simulink model "XY_2_pen_ros2"  (R2024b)
settings: Solver=ode4  StartTime=0.0  StopTime=T_run_ros  FixedStep=Ts_ctrl  RelTol=1e-3
StopFcn:
  | XY_stop
values from neighbouring files (symbols this model uses):
  d_reach = 0.03    [XY_setup.m]
  db_v = 47    [XY_setup.m]
  db_w = 20    [XY_setup.m]
  K_c = 0    [XY_setup.m]
  K_ci = 0    [XY_setup.m]
  K_dist = 1.0    (= 1)    [XY_setup.m]
  K_ptheta = 1.4    [XY_setup.m]
  K_px = 0.3    [XY_setup.m]
  K_py = 5.0    (= 5)    [XY_setup.m]
  K_yaw = 2.0    (= 2)    [XY_setup.m]
  line_post = 0.04    [XY_setup.m]
  line_pre = 0.06    [XY_setup.m]
  pen_A = [-0.70; 0.30]    [XY_setup.m]
  pen_B = [ 0.50; 0.30]    [XY_setup.m]
  pen_d = r_pen0 - r_tag    [XY_setup.m]
  psi0 = pi/2    (= 1.57079632679)    [XY_setup.m]
  r_tag = [-0.080;  0.060]    [XY_setup.m]
  stage_c = stage_travel/2    (= 50.8)    [XY_setup.m]
  stage_travel = 101.6    [XY_setup.m]
  stage_vcmd = 0.8*stage_vmax    (= 83.2)    [XY_setup.m]
  tau_pred = 0    [XY_setup.m]
  th_tol = deg2rad(1)    [XY_setup.m]
  Ts_ctrl = 0.01    [XY_setup.m]
  v_full = 0.20    (= 0.2)    [XY_setup.m]
  v_max = 0.20    (= 0.2)    [XY_setup.m]
  v_ref = 0.03    [XY_setup.m]
  w_full = 2*k_pwm*(400 - db_w)/B_eff    (= 1.36936936937)    [XY_setup.m]
  w_max = deg2rad(45)    [XY_setup.m]
  x = c(1) + s(1)/2*[-1 1 1 -1 -1 1 1 -1]    [XY_animate.m]
  y = c(2) + s(2)/2*[-1 -1 1 1 -1 -1 1 1]    [XY_animate.m]    (also in build_xy_models.m = q(2))
  zk_xsign = -1    [XY_setup.m]
libraries: ros2lib x8, simulink x4
settings Model: Creator=admin  LastModifiedBy=admin
settings DataIOCC: ReturnWorkspaceOutputs=off

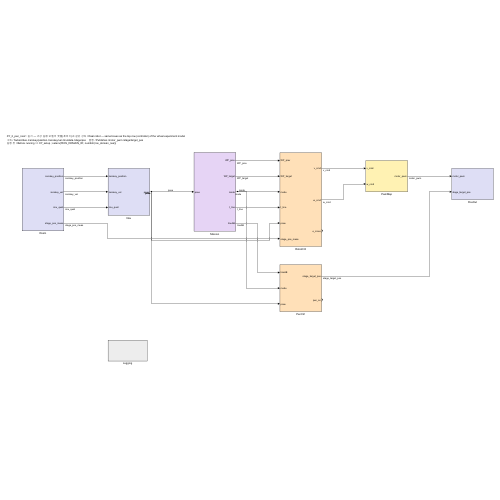
[thumbnail: Simulink's stored preview of the top-level diagram]
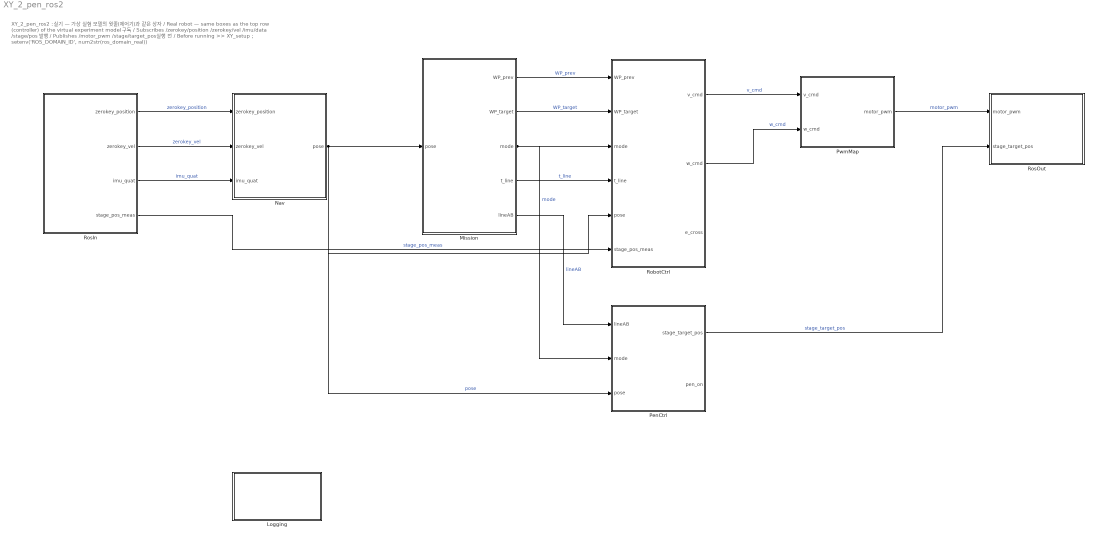
== system XY_2_pen_ros2 ==
  note: XY_2_pen_ros2 : 실기 — 가상 실험 모델의 윗줄(제어기)과 같은 상자 / Real robot — same boxes as the top row (controller) of the virtual experiment model
      | 구독 / Subscribes /zerokey/position /zerokey/vel /imu/data /stage/pos    발행 / Publishes /motor_pwm /stage/target_pos
      | 실행 전 / Before running >> XY_setup ; setenv('ROS_DOMAIN_ID', num2str(ros_domain_real))
  Logging : Subsystem
  Mission : Subsystem
  Nav : Subsystem
  PenCtrl : Subsystem
  PwmMap : Subsystem
  RobotCtrl : Subsystem
  RosIn : Subsystem
  RosOut : Subsystem
  wires:
  Nav/1(pose) -> Mission/1(pose), PenCtrl/3(pose), RobotCtrl/5(pose)  "pose"
  RosIn/1(zerokey_position) -> Nav/1(zerokey_position)  "zerokey_position"
  RosIn/2(zerokey_vel) -> Nav/2(zerokey_vel)  "zerokey_vel"
  RosIn/3(imu_quat) -> Nav/3(imu_quat)  "imu_quat"
  Mission/5(lineAB) -> PenCtrl/1(lineAB)  "lineAB"
  Mission/3(mode) -> PenCtrl/2(mode), RobotCtrl/3(mode)  "mode"
  RobotCtrl/1(v_cmd) -> PwmMap/1(v_cmd)  "v_cmd"
  RobotCtrl/2(w_cmd) -> PwmMap/2(w_cmd)  "w_cmd"
  Mission/1(WP_prev) -> RobotCtrl/1(WP_prev)  "WP_prev"
  Mission/2(WP_target) -> RobotCtrl/2(WP_target)  "WP_target"
  Mission/4(t_line) -> RobotCtrl/4(t_line)  "t_line"
  RosIn/4(stage_pos_meas) -> RobotCtrl/6(stage_pos_meas)  "stage_pos_meas"
  PwmMap/1(motor_pwm) -> RosOut/1(motor_pwm)  "motor_pwm"
  PenCtrl/1(stage_target_pos) -> RosOut/2(stage_target_pos)  "stage_target_pos"

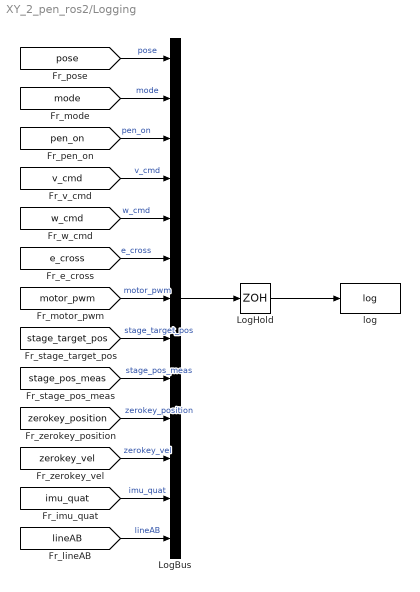
== system XY_2_pen_ros2/Logging ==
  LogBus : BusCreator  Inputs=13
  LogHold : ZeroOrderHold  Description=이산: 기록 주기 (제어기 주기와 같다) / Discrete: logging period (same as the controller period)  SampleTime=Ts_ctrl
  log : ToWorkspace  VariableName=log  SaveFormat=Timeseries  SampleTime=Ts_ctrl
  wires:
  [pose] -> LogBus/1  "pose"
  [mode] -> LogBus/2  "mode"
  [pen_on] -> LogBus/3  "pen_on"
  [v_cmd] -> LogBus/4  "v_cmd"
  [w_cmd] -> LogBus/5  "w_cmd"
  [e_cross] -> LogBus/6  "e_cross"
  [motor_pwm] -> LogBus/7  "motor_pwm"
  [stage_target_pos] -> LogBus/8  "stage_target_pos"
  [stage_pos_meas] -> LogBus/9  "stage_pos_meas"
  [zerokey_position] -> LogBus/10  "zerokey_position"
  [zerokey_vel] -> LogBus/11  "zerokey_vel"
  [imu_quat] -> LogBus/12  "imu_quat"
  [lineAB] -> LogBus/13  "lineAB"
  LogBus/1 -> LogHold/1
  LogHold/1 -> log/1

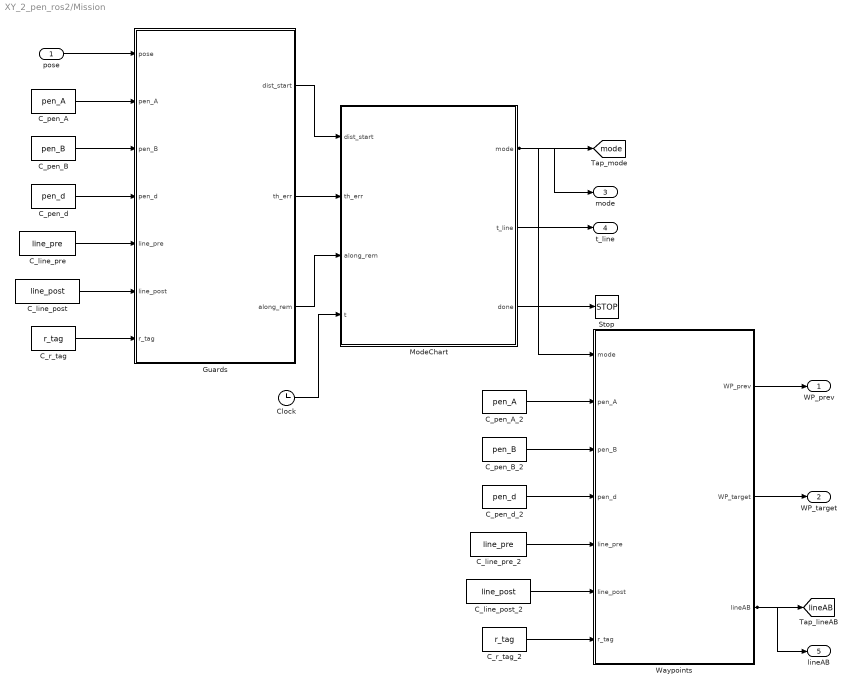
== system XY_2_pen_ros2/Mission ==
  pose : Inport
  C_line_post : Constant  Value=line_post
  C_line_post_2 : Constant  Value=line_post
  C_line_pre : Constant  Value=line_pre
  C_line_pre_2 : Constant  Value=line_pre
  C_pen_A : Constant  Value=pen_A
  C_pen_A_2 : Constant  Value=pen_A
  C_pen_B : Constant  Value=pen_B
  C_pen_B_2 : Constant  Value=pen_B
  C_pen_d : Constant  Value=pen_d
  C_pen_d_2 : Constant  Value=pen_d
  C_r_tag : Constant  Value=r_tag
  C_r_tag_2 : Constant  Value=r_tag
  Clock : Clock
  Guards : MATLAB Function  TreatAsAtomicUnit=on
  ModeChart : Stateflow chart  Description=이산: 모드는 사건 상태 (6WP_sim Chart 와 같은 역할). 전이: 거리 < d_reach, 1 s 뒤 각 오차 < th_tol, 남은 거리 < d_reach, 정지 2 s / Discrete: the mode is an event state (same role as the 6WP_sim Chart). Transitions: distance < d_reach, angle error < th_tol after 1 s, remaining distance < d_reach, stop 2 s  TreatAsAtomicUnit=on
  Stop : Stop
  Waypoints : MATLAB Function  TreatAsAtomicUnit=on
  WP_prev : Outport
  WP_target : Outport  Port=2
  mode : Outport  Port=3
  t_line : Outport  Port=4
  lineAB : Outport  Port=5
  tag scope: lineAB=global, mode=global
  wires:
  pose/1 -> Guards/1(pose)
  Clock/1 -> ModeChart/4(t)
  C_pen_A/1 -> Guards/2(pen_A)
  C_pen_d/1 -> Guards/4(pen_d)
  C_pen_B/1 -> Guards/3(pen_B)
  C_line_pre/1 -> Guards/5(line_pre)
  C_line_post/1 -> Guards/6(line_post)
  C_r_tag/1 -> Guards/7(r_tag)
  Guards/1(dist_start) -> ModeChart/1(dist_start)
  Guards/2(th_err) -> ModeChart/2(th_err)
  Guards/3(along_rem) -> ModeChart/3(along_rem)
  ModeChart/1(mode) -> Waypoints/1(mode), mode/1, [mode]
  ModeChart/2(t_line) -> t_line/1
  ModeChart/3(done) -> Stop/1
  C_pen_A_2/1 -> Waypoints/2(pen_A)
  C_pen_B_2/1 -> Waypoints/3(pen_B)
  C_pen_d_2/1 -> Waypoints/4(pen_d)
  C_line_pre_2/1 -> Waypoints/5(line_pre)
  C_line_post_2/1 -> Waypoints/6(line_post)
  C_r_tag_2/1 -> Waypoints/7(r_tag)
  Waypoints/1(WP_prev) -> WP_prev/1
  Waypoints/2(WP_target) -> WP_target/1
  Waypoints/3(lineAB) -> lineAB/1, [lineAB]

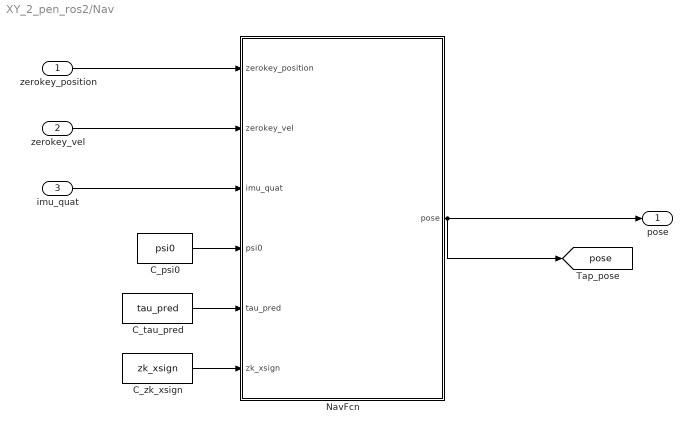
== system XY_2_pen_ros2/Nav ==
  zerokey_position : Inport
  zerokey_vel : Inport  Port=2
  imu_quat : Inport  Port=3
  C_psi0 : Constant  Value=psi0
  C_tau_pred : Constant  Value=tau_pred
  C_zk_xsign : Constant  Value=zk_xsign
  NavFcn : MATLAB Function  Description=이산: persistent (첫 요각 기억) — 구독 주기와 같다 / Discrete: persistent (stores the first yaw) — same as the subscription period  TreatAsAtomicUnit=on
  pose : Outport
  tag scope: pose=global
  wires:
  zerokey_position/1 -> NavFcn/1(zerokey_position)
  zerokey_vel/1 -> NavFcn/2(zerokey_vel)
  imu_quat/1 -> NavFcn/3(imu_quat)
  C_psi0/1 -> NavFcn/4(psi0)
  C_tau_pred/1 -> NavFcn/5(tau_pred)
  C_zk_xsign/1 -> NavFcn/6(zk_xsign)
  NavFcn/1(pose) -> pose/1, [pose]

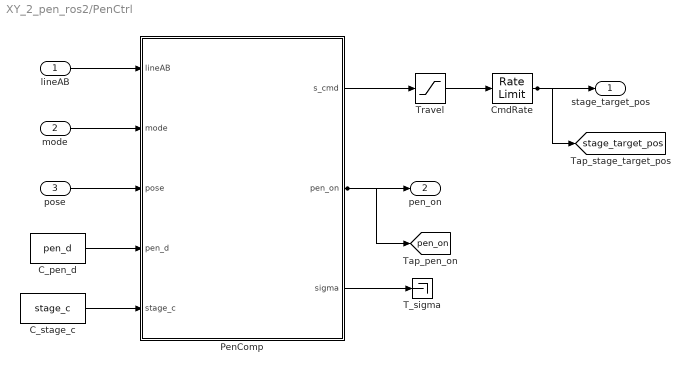
== system XY_2_pen_ros2/PenCtrl ==
  lineAB : Inport
  mode : Inport  Port=2
  pose : Inport  Port=3
  C_pen_d : Constant  Value=pen_d
  C_stage_c : Constant  Value=stage_c
  CmdRate : RateLimiter  RisingSlewLimit=stage_vcmd  FallingSlewLimit=-stage_vcmd  SampleTimeMode=inherited  InitialCondition=stage_c
  PenComp : MATLAB Function  TreatAsAtomicUnit=on
  T_sigma : Terminator
  Travel : Saturate  UpperLimit=stage_travel  LowerLimit=0
  stage_target_pos : Outport
  pen_on : Outport  Port=2
  tag scope: pen_on=global, stage_target_pos=global
  wires:
  PenComp/3(sigma) -> T_sigma/1
  lineAB/1 -> PenComp/1(lineAB)
  C_stage_c/1 -> PenComp/5(stage_c)
  C_pen_d/1 -> PenComp/4(pen_d)
  mode/1 -> PenComp/2(mode)
  PenComp/2(pen_on) -> pen_on/1, [pen_on]
  Travel/1 -> CmdRate/1
  pose/1 -> PenComp/3(pose)
  PenComp/1(s_cmd) -> Travel/1
  CmdRate/1 -> stage_target_pos/1, [stage_target_pos]

== system XY_2_pen_ros2/PwmMap ==
  v_cmd : Inport
  w_cmd : Inport  Port=2
  C_db_v : Constant  Value=db_v
  C_db_w : Constant  Value=db_w
  C_v_full : Constant  Value=v_full
  C_w_full : Constant  Value=w_full
  calc_pwm : MATLAB Function  TreatAsAtomicUnit=on
  motor_pwm : Outport
  tag scope: motor_pwm=global
  wires:
  v_cmd/1 -> calc_pwm/1(v_cmd)
  w_cmd/1 -> calc_pwm/2(w_cmd)
  C_v_full/1 -> calc_pwm/3(v_full)
  C_w_full/1 -> calc_pwm/4(w_full)
  C_db_v/1 -> calc_pwm/5(db_v)
  C_db_w/1 -> calc_pwm/6(db_w)
  calc_pwm/1(motor_pwm) -> motor_pwm/1, [motor_pwm]

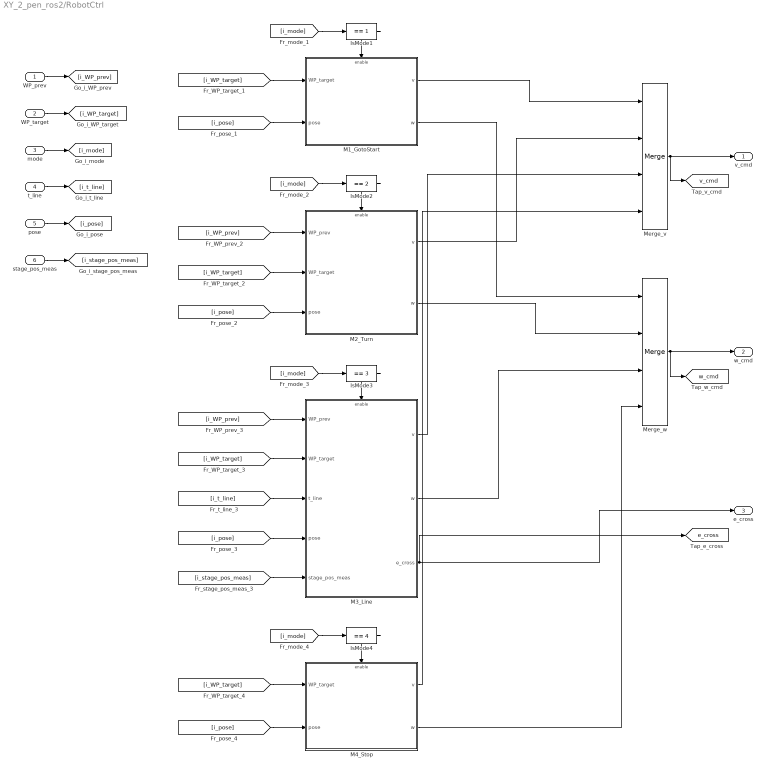
== system XY_2_pen_ros2/RobotCtrl ==
  WP_prev : Inport
  WP_target : Inport  Port=2
  mode : Inport  Port=3
  t_line : Inport  Port=4
  pose : Inport  Port=5
  stage_pos_meas : Inport  Port=6
  IsMode1 : simulink/Logic and Bit Operations/Compare To Constant  relop===  const=1  OutDataTypeStr=boolean
  IsMode2 : simulink/Logic and Bit Operations/Compare To Constant  relop===  const=2  OutDataTypeStr=boolean
  IsMode3 : simulink/Logic and Bit Operations/Compare To Constant  relop===  const=3  OutDataTypeStr=boolean
  IsMode4 : simulink/Logic and Bit Operations/Compare To Constant  relop===  const=4  OutDataTypeStr=boolean
  M1_GotoStart : Subsystem
  M2_Turn : Subsystem
  M3_Line : Subsystem
  M4_Stop : Subsystem
  Merge_v : Merge  Inputs=4
  Merge_w : Merge  Inputs=4
  v_cmd : Outport
  w_cmd : Outport  Port=2
  e_cross : Outport  Port=3
  tag scope: e_cross=global, v_cmd=global, w_cmd=global
  wires:
  WP_prev/1 -> [i_WP_prev]
  WP_target/1 -> [i_WP_target]
  mode/1 -> [i_mode]
  t_line/1 -> [i_t_line]
  pose/1 -> [i_pose]
  stage_pos_meas/1 -> [i_stage_pos_meas]
  [i_WP_target] -> M1_GotoStart/1(WP_target)
  [i_pose] -> M1_GotoStart/2(pose)
  [i_mode] -> IsMode1/1
  IsMode1/1 -> M1_GotoStart/Enable
  [i_WP_prev] -> M2_Turn/1(WP_prev)
  [i_WP_target] -> M2_Turn/2(WP_target)
  [i_pose] -> M2_Turn/3(pose)
  [i_mode] -> IsMode2/1
  IsMode2/1 -> M2_Turn/Enable
  [i_WP_prev] -> M3_Line/1(WP_prev)
  [i_WP_target] -> M3_Line/2(WP_target)
  [i_t_line] -> M3_Line/3(t_line)
  [i_pose] -> M3_Line/4(pose)
  [i_stage_pos_meas] -> M3_Line/5(stage_pos_meas)
  [i_mode] -> IsMode3/1
  IsMode3/1 -> M3_Line/Enable
  [i_WP_target] -> M4_Stop/1(WP_target)
  [i_pose] -> M4_Stop/2(pose)
  [i_mode] -> IsMode4/1
  IsMode4/1 -> M4_Stop/Enable
  Merge_v/1 -> v_cmd/1, [v_cmd]
  Merge_w/1 -> w_cmd/1, [w_cmd]
  M3_Line/3(e_cross) -> e_cross/1, [e_cross]
  M1_GotoStart/1(v) -> Merge_v/1
  M2_Turn/1(v) -> Merge_v/2
  M3_Line/1(v) -> Merge_v/3
  M4_Stop/1(v) -> Merge_v/4
  M1_GotoStart/2(w) -> Merge_w/1
  M2_Turn/2(w) -> Merge_w/2
  M3_Line/2(w) -> Merge_w/3
  M4_Stop/2(w) -> Merge_w/4

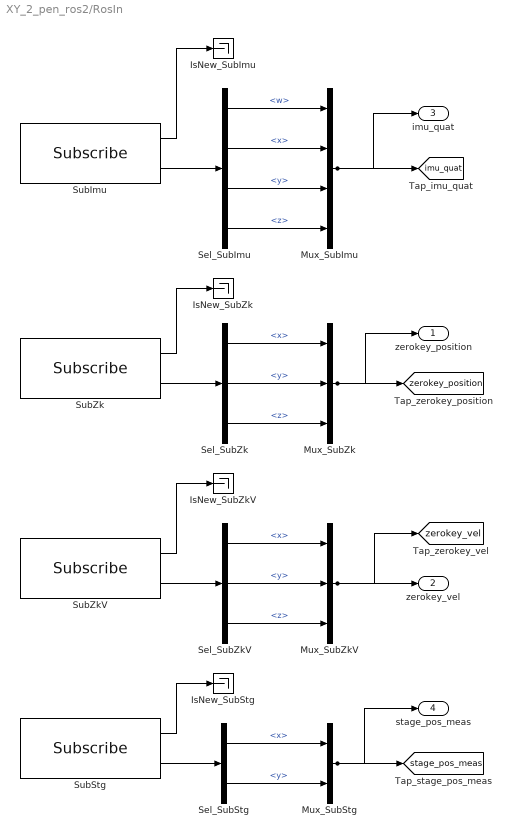
== system XY_2_pen_ros2/RosIn ==
  IsNew_SubImu : Terminator
  IsNew_SubStg : Terminator
  IsNew_SubZk : Terminator
  IsNew_SubZkV : Terminator
  Mux_SubImu : Mux
  Mux_SubStg : Mux  Inputs=2
  Mux_SubZk : Mux  Inputs=3
  Mux_SubZkV : Mux  Inputs=3
  Sel_SubImu : BusSelector  OutputSignals=orientation.w,orientation.x,orientation.y,orientation.z
  Sel_SubStg : BusSelector  OutputSignals=point.x,point.y
  Sel_SubZk : BusSelector  OutputSignals=point.x,point.y,point.z
  Sel_SubZkV : BusSelector  OutputSignals=twist.linear.x,twist.linear.y,twist.linear.z
  SubImu : ros2lib/Subscribe  Description=이산: ROS Subscribe 는 구독 주기로만 돈다 / Discrete: ROS Subscribe runs only at the subscription period  topicSource=Specify your own  topic=/imu/data  messageType=sensor_msgs/Imu  sampleTime=Ts_ctrl  QOSHistory=Keep last  QOSDepth=1  QOSReliability=Reliable  QOSDurability=Volatile  QOSDeadline=Inf  QOSLifespan=Inf  QOSLiveliness=Automatic  QOSLeaseDuration=Inf  QOSAvoidROSNamespaceConventions=off
  SubStg : ros2lib/Subscribe  Description=이산: ROS Subscribe 는 구독 주기로만 돈다 / Discrete: ROS Subscribe runs only at the subscription period  topicSource=Specify your own  topic=/stage/pos  messageType=geometry_msgs/PointStamped  sampleTime=Ts_ctrl  QOSHistory=Keep last  QOSDepth=1  QOSReliability=Reliable  QOSDurability=Volatile  QOSDeadline=Inf  QOSLifespan=Inf  QOSLiveliness=Automatic  QOSLeaseDuration=Inf  QOSAvoidROSNamespaceConventions=off
  SubZk : ros2lib/Subscribe  Description=이산: ROS Subscribe 는 구독 주기로만 돈다 / Discrete: ROS Subscribe runs only at the subscription period  topicSource=Specify your own  topic=/zerokey/position  messageType=geometry_msgs/PointStamped  sampleTime=Ts_ctrl  QOSHistory=Keep last  QOSDepth=1  QOSReliability=Reliable  QOSDurability=Volatile  QOSDeadline=Inf  QOSLifespan=Inf  QOSLiveliness=Automatic  QOSLeaseDuration=Inf  QOSAvoidROSNamespaceConventions=off
  SubZkV : ros2lib/Subscribe  Description=이산: ROS Subscribe 는 구독 주기로만 돈다 / Discrete: ROS Subscribe runs only at the subscription period  topicSource=Specify your own  topic=/zerokey/vel  messageType=geometry_msgs/TwistStamped  sampleTime=Ts_ctrl  QOSHistory=Keep last  QOSDepth=1  QOSReliability=Reliable  QOSDurability=Volatile  QOSDeadline=Inf  QOSLifespan=Inf  QOSLiveliness=Automatic  QOSLeaseDuration=Inf  QOSAvoidROSNamespaceConventions=off
  zerokey_position : Outport
  zerokey_vel : Outport  Port=2
  imu_quat : Outport  Port=3
  stage_pos_meas : Outport  Port=4
  tag scope: imu_quat=global, stage_pos_meas=global, zerokey_position=global, zerokey_vel=global
  wires:
  Sel_SubStg/2 -> Mux_SubStg/2  "<y>"
  SubStg/2 -> Sel_SubStg/1
  Sel_SubZk/2 -> Mux_SubZk/2  "<y>"
  SubImu/1 -> IsNew_SubImu/1
  Sel_SubZk/3 -> Mux_SubZk/3  "<z>"
  SubZkV/1 -> IsNew_SubZkV/1
  SubImu/2 -> Sel_SubImu/1
  SubZkV/2 -> Sel_SubZkV/1
  Sel_SubZkV/3 -> Mux_SubZkV/3  "<z>"
  Sel_SubImu/2 -> Mux_SubImu/2  "<x>"
  SubZk/1 -> IsNew_SubZk/1
  Mux_SubZkV/1 -> zerokey_vel/1, [zerokey_vel]
  SubStg/1 -> IsNew_SubStg/1
  SubZk/2 -> Sel_SubZk/1
  Sel_SubZkV/2 -> Mux_SubZkV/2  "<y>"
  Sel_SubImu/1 -> Mux_SubImu/1  "<w>"
  Sel_SubImu/3 -> Mux_SubImu/3  "<y>"
  Sel_SubImu/4 -> Mux_SubImu/4  "<z>"
  Sel_SubZk/1 -> Mux_SubZk/1  "<x>"
  Sel_SubZkV/1 -> Mux_SubZkV/1  "<x>"
  Sel_SubStg/1 -> Mux_SubStg/1  "<x>"
  Mux_SubImu/1 -> imu_quat/1, [imu_quat]
  Mux_SubZk/1 -> zerokey_position/1, [zerokey_position]
  Mux_SubStg/1 -> stage_pos_meas/1, [stage_pos_meas]

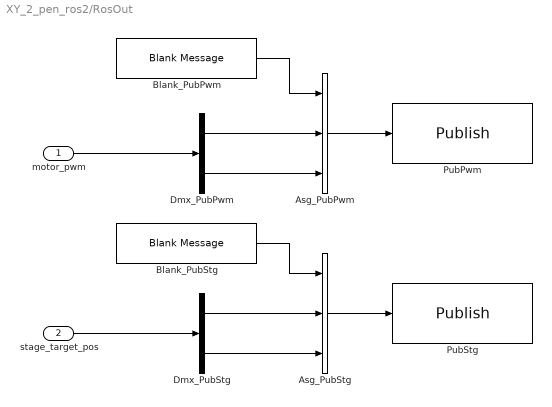
== system XY_2_pen_ros2/RosOut ==
  motor_pwm : Inport
  stage_target_pos : Inport  Port=2
  Asg_PubPwm : BusAssignment  AssignedSignals=x,y
  Asg_PubStg : BusAssignment  AssignedSignals=x,y
  Blank_PubPwm : ros2lib/Blank Message  messageClass=Message  entityType=geometry_msgs/Point  messageType=geometry_msgs/Point  SampleTime=inf
  Blank_PubStg : ros2lib/Blank Message  messageClass=Message  entityType=geometry_msgs/Point  messageType=geometry_msgs/Point  SampleTime=inf
  Dmx_PubPwm : Demux  Outputs=2
  Dmx_PubStg : Demux  Outputs=2
  PubPwm : ros2lib/Publish  topicSource=Specify your own  topic=/motor_pwm  messageType=geometry_msgs/Point  QOSHistory=Keep last  QOSDepth=1  QOSReliability=Reliable  QOSDurability=Volatile  QOSDeadline=Inf  QOSLifespan=Inf  QOSLiveliness=Automatic  QOSLeaseDuration=Inf  QOSAvoidROSNamespaceConventions=off
  PubStg : ros2lib/Publish  topicSource=Specify your own  topic=/stage/target_pos  messageType=geometry_msgs/Point  QOSHistory=Keep last  QOSDepth=1  QOSReliability=Reliable  QOSDurability=Volatile  QOSDeadline=Inf  QOSLifespan=Inf  QOSLiveliness=Automatic  QOSLeaseDuration=Inf  QOSAvoidROSNamespaceConventions=off
  wires:
  Blank_PubStg/1 -> Asg_PubStg/1
  Dmx_PubPwm/2 -> Asg_PubPwm/3
  motor_pwm/1 -> Dmx_PubPwm/1
  Blank_PubPwm/1 -> Asg_PubPwm/1
  stage_target_pos/1 -> Dmx_PubStg/1
  Dmx_PubPwm/1 -> Asg_PubPwm/2
  Dmx_PubStg/1 -> Asg_PubStg/2
  Dmx_PubStg/2 -> Asg_PubStg/3
  Asg_PubPwm/1 -> PubPwm/1
  Asg_PubStg/1 -> PubStg/1

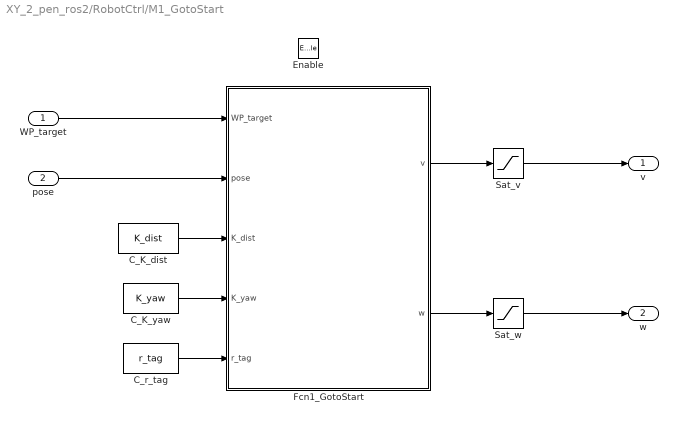
== system XY_2_pen_ros2/RobotCtrl/M1_GotoStart ==
  WP_target : Inport
  pose : Inport  Port=2
  Enable : EnablePort
  C_K_dist : Constant  Value=K_dist
  C_K_yaw : Constant  Value=K_yaw
  C_r_tag : Constant  Value=r_tag
  Fcn1_GotoStart : MATLAB Function  TreatAsAtomicUnit=on
  Sat_v : Saturate  UpperLimit=v_max  LowerLimit=-(v_max)
  Sat_w : Saturate  UpperLimit=w_max  LowerLimit=-(w_max)
  v : Outport
  w : Outport  Port=2
  wires:
  WP_target/1 -> Fcn1_GotoStart/1(WP_target)
  pose/1 -> Fcn1_GotoStart/2(pose)
  C_K_dist/1 -> Fcn1_GotoStart/3(K_dist)
  C_K_yaw/1 -> Fcn1_GotoStart/4(K_yaw)
  C_r_tag/1 -> Fcn1_GotoStart/5(r_tag)
  Fcn1_GotoStart/1(v) -> Sat_v/1
  Sat_v/1 -> v/1
  Fcn1_GotoStart/2(w) -> Sat_w/1
  Sat_w/1 -> w/1

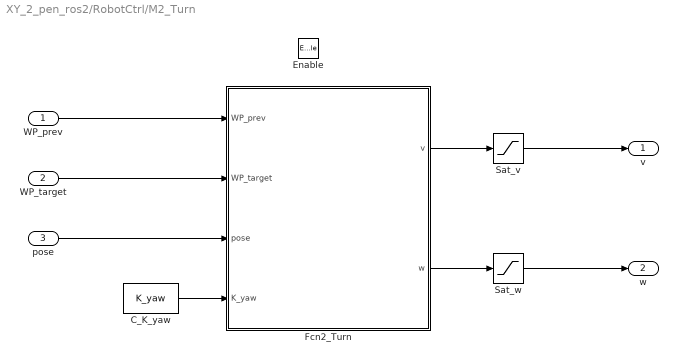
== system XY_2_pen_ros2/RobotCtrl/M2_Turn ==
  WP_prev : Inport
  WP_target : Inport  Port=2
  pose : Inport  Port=3
  Enable : EnablePort
  C_K_yaw : Constant  Value=K_yaw
  Fcn2_Turn : MATLAB Function  TreatAsAtomicUnit=on
  Sat_v : Saturate  UpperLimit=v_max  LowerLimit=-(v_max)
  Sat_w : Saturate  UpperLimit=w_max  LowerLimit=-(w_max)
  v : Outport
  w : Outport  Port=2
  wires:
  WP_prev/1 -> Fcn2_Turn/1(WP_prev)
  WP_target/1 -> Fcn2_Turn/2(WP_target)
  pose/1 -> Fcn2_Turn/3(pose)
  C_K_yaw/1 -> Fcn2_Turn/4(K_yaw)
  Fcn2_Turn/1(v) -> Sat_v/1
  Sat_v/1 -> v/1
  Fcn2_Turn/2(w) -> Sat_w/1
  Sat_w/1 -> w/1

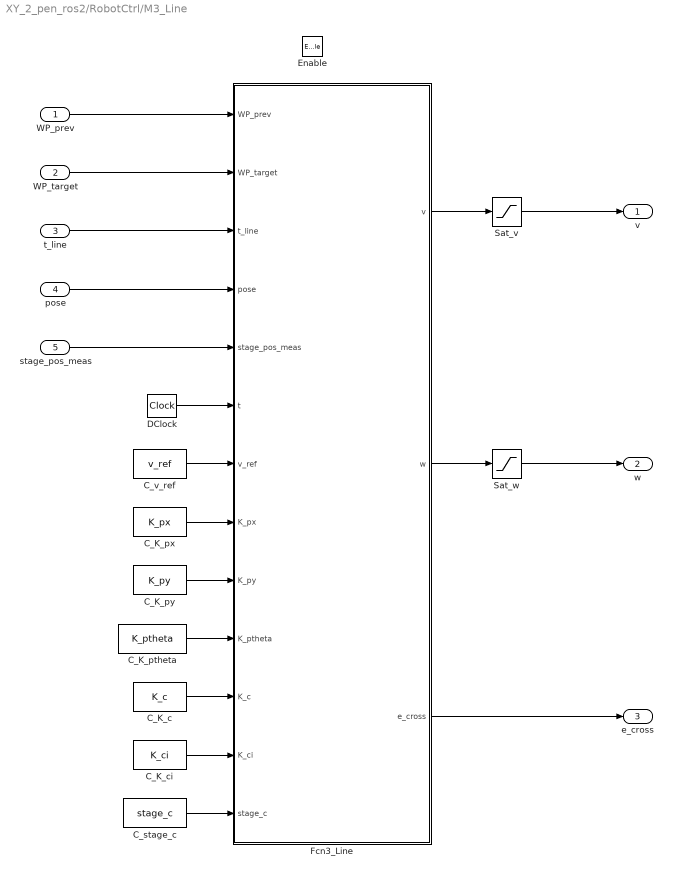
== system XY_2_pen_ros2/RobotCtrl/M3_Line ==
  WP_prev : Inport
  WP_target : Inport  Port=2
  t_line : Inport  Port=3
  pose : Inport  Port=4
  stage_pos_meas : Inport  Port=5
  Enable : EnablePort
  C_K_c : Constant  Value=K_c
  C_K_ci : Constant  Value=K_ci
  C_K_ptheta : Constant  Value=K_ptheta
  C_K_px : Constant  Value=K_px
  C_K_py : Constant  Value=K_py
  C_stage_c : Constant  Value=stage_c
  C_v_ref : Constant  Value=v_ref
  DClock : DigitalClock  Description=이산: 제어기 주기의 시간 (Merge 앞 모드 상자 샘플 시간 통일) / Discrete: time at the controller period (common sample time for the mode boxes before Merge)  SampleTime=Ts_ctrl
  Fcn3_Line : MATLAB Function  TreatAsAtomicUnit=on
  Sat_v : Saturate  UpperLimit=v_max  LowerLimit=-(v_max)
  Sat_w : Saturate  UpperLimit=w_max  LowerLimit=-(w_max)
  v : Outport
  w : Outport  Port=2
  e_cross : Outport  Port=3
  wires:
  WP_prev/1 -> Fcn3_Line/1(WP_prev)
  WP_target/1 -> Fcn3_Line/2(WP_target)
  t_line/1 -> Fcn3_Line/3(t_line)
  pose/1 -> Fcn3_Line/4(pose)
  stage_pos_meas/1 -> Fcn3_Line/5(stage_pos_meas)
  DClock/1 -> Fcn3_Line/6(t)
  C_v_ref/1 -> Fcn3_Line/7(v_ref)
  C_K_px/1 -> Fcn3_Line/8(K_px)
  C_K_py/1 -> Fcn3_Line/9(K_py)
  C_K_ptheta/1 -> Fcn3_Line/10(K_ptheta)
  C_K_c/1 -> Fcn3_Line/11(K_c)
  C_K_ci/1 -> Fcn3_Line/12(K_ci)
  C_stage_c/1 -> Fcn3_Line/13(stage_c)
  Fcn3_Line/1(v) -> Sat_v/1
  Sat_v/1 -> v/1
  Fcn3_Line/2(w) -> Sat_w/1
  Sat_w/1 -> w/1
  Fcn3_Line/3(e_cross) -> e_cross/1

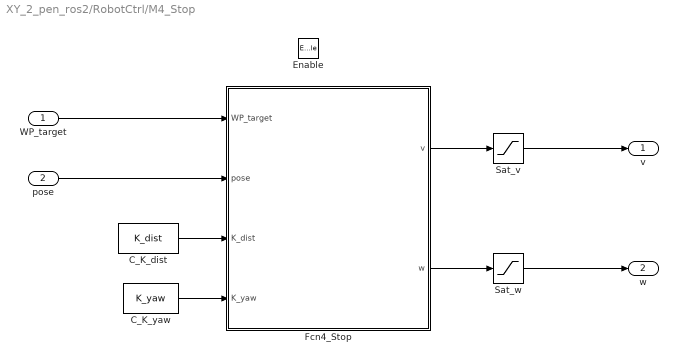
== system XY_2_pen_ros2/RobotCtrl/M4_Stop ==
  WP_target : Inport
  pose : Inport  Port=2
  Enable : EnablePort
  C_K_dist : Constant  Value=K_dist
  C_K_yaw : Constant  Value=K_yaw
  Fcn4_Stop : MATLAB Function  TreatAsAtomicUnit=on
  Sat_v : Saturate  UpperLimit=v_max  LowerLimit=-(v_max)
  Sat_w : Saturate  UpperLimit=w_max  LowerLimit=-(w_max)
  v : Outport
  w : Outport  Port=2
  wires:
  WP_target/1 -> Fcn4_Stop/1(WP_target)
  pose/1 -> Fcn4_Stop/2(pose)
  C_K_dist/1 -> Fcn4_Stop/3(K_dist)
  C_K_yaw/1 -> Fcn4_Stop/4(K_yaw)
  Fcn4_Stop/1(v) -> Sat_v/1
  Sat_v/1 -> v/1
  Fcn4_Stop/2(w) -> Sat_w/1
  Sat_w/1 -> w/1

== matlab function XY_2_pen_ros2/RobotCtrl/M3_Line/Fcn3_Line ==
  data: WP_prev input; v output; WP_target input; t_line input; pose input; stage_pos_meas input; t input; v_ref input; K_px input; K_py input; K_ptheta input; K_c input; K_ci input; stage_c input; w output; e_cross output
function [v, w, e_cross] = Line_Tracking_Mode(WP_prev, WP_target, t_line, pose, stage_pos_meas, t, v_ref, K_px, K_py, K_ptheta, K_c, K_ci, stage_c)
% 모드 3 : 6WP_sim Line_Tracking_Mode — 시간에 따라 앞서 가는 기준점 + 바디 좌표 오차 (게인은 실기 ZeroKey 모델 값)
% Mode 3 : 6WP_sim Line_Tracking_Mode — time-parameterised reference point + body-frame error (real ZeroKey model gains)
% 입력 / Inputs
%   WP_prev, WP_target [2x1, m]  태그 선분 rA -> rB / tag segment
%   t_line [s]  모드 3 진입 시각 / time mode 3 started;   t [s] 현재 시각 / current time
%   pose   [3x1: m, m, rad]  측정 태그 자세 / measured tag pose
%   stage_pos_meas [2x1, mm] /stage/pos (K_c = K_ci = 0 이면 쓰지 않음 / unused when K_c = K_ci = 0)
%   v_ref [m/s] 직선 속도 / line speed;  K_px [1/s];  K_py [rad/(m s)];  K_ptheta [1/s]
%   K_c [-] 스테이지 중앙 유지 비례 / stage-centring P;  K_ci [1/s] 그 적분 / its integral;  stage_c [mm] 스테이지 중앙 / stage centre
% 출력 / Outputs
%   v [m/s], w [rad/s]  속도 명령 / speed commands;   e_cross [m]  바디 좌표 횡오차 e_y / body-frame cross error
% 원리 / Principle
%   x_r = rA + v_ref (t - t_line) u,  [e_x; e_y] = R(psi)^T (x_r - p),  e_th = theta_l - psi
%   v = v_ref cos e_th + K_px e_x,  w = K_py e_y + K_ptheta sin e_th
%   로봇은 옆으로 못 가므로 횡오차 e_y 는 회전(w)으로만 줄인다 / a tracked robot cannot slide sideways, so e_y is removed by turning
th_final = atan2(WP_target(2) - WP_prev(2), WP_target(1) - WP_prev(1));
dist_total = hypot(WP_target(1) - WP_prev(1), WP_target(2) - WP_prev(2));
d_traj = min(v_ref * (t - t_line), dist_total);
x_r = WP_prev(1) + d_traj * cos(th_final);
y_r = WP_prev(2) + d_traj * sin(th_final);
if d_traj < dist_total, vr = v_ref; else, vr = 0; end
theta = pose(3);
err_g = [x_r - pose(1); y_r - pose(2); th_final - theta];
R_mat = [cos(theta) sin(theta) 0; -sin(theta) cos(theta) 0; 0 0 1];
ep = R_mat * err_g;
eth = atan2(sin(ep(3)), cos(ep(3)));
e_cross = ep(2);
v = vr * cos(eth) + K_px * ep(1);
% 스테이지 중앙 유지 (K_c = 0 이면 끔): 스테이지 Y 가 중앙에서 벗어난 만큼을 횡오차에 더해
% 로봇이 펜 쪽으로 다가가게 한다 -> 스테이지가 행정 가운데에서 일한다
% Stage centring (off when K_c = 0): the stage Y offset from centre is added to the cross error
% so the robot moves toward the pen -> the stage works in the middle of its travel
%   비례(K_c) + 적분(K_ci): 적분이 벽면 미끄러짐으로 생기는 정상 편차를 없앤다
%   P (K_c) + I (K_ci): the integral removes the steady offset caused by slip on the wall
persistent I t_prev
if isempty(I), I = 0; t_prev = t; end
e_s = (stage_pos_meas(2) - stage_c) / 1000;   % 스테이지 Y 편차 [m] / stage Y offset [m]
I = I + K_ci * e_s * max(t - t_prev, 0);  t_prev = t;
e_c = ep(2) + K_c * e_s + I;
w = K_py * e_c + K_ptheta * sin(eth);

== matlab function XY_2_pen_ros2/RobotCtrl/M4_Stop/Fcn4_Stop ==
  data: WP_target input; v output; pose input; K_dist input; K_yaw input; w output
function [v, w] = Stop_Destination_Mode(WP_target, pose, K_dist, K_yaw)
% 모드 4 : 6WP_sim Stop_Destination_Mode — 끝점(WP_target) 으로 Goto 식을 계속 돌려 그 자리에 머문다
% Mode 4 : 6WP_sim Stop_Destination_Mode — keeps running the go-to law on the end point to hold position
% 입력 / Inputs : WP_target = rB [2x1, m], pose [m, m, rad], K_dist [1/s], K_yaw [1/s]
% 출력 / Outputs: v [m/s], w [rad/s]  (끝점 10 mm 안에서는 w = 0 / w = 0 within 10 mm of the end point)
err_x = WP_target(1) - pose(1);  err_y = WP_target(2) - pose(2);
dist = hypot(err_x, err_y);
target_th = atan2(err_y, err_x);
a = atan2(sin(target_th - pose(3)), cos(target_th - pose(3)));
v = K_dist * dist * max(0, cos(a));
w = K_yaw * a + 0.5 * sin(a) * cos(a);
if dist < 0.01, w = 0; end                     % 끝점 위에서는 방향을 돌리지 않는다 / no turning on the end point

== matlab function XY_2_pen_ros2/PwmMap/calc_pwm ==
  data: v_cmd input; motor_pwm output; w_cmd input; v_full input; w_full input; db_v input; db_w input
function motor_pwm = calc_pwm(v_cmd, w_cmd, v_full, w_full, db_v, db_w)
% calc_pwm : 차체 속도 명령 -> 좌우 모터 PWM (실기 MATLAB Function6 calc_pwm 과 같은 식)
% calc_pwm : body speed command -> left/right motor PWM (same as the real MATLAB Function6 calc_pwm)
% 입력 / Inputs
%   v_cmd  [m/s]    전진 속도 명령 (RobotCtrl) / forward speed command
%   w_cmd  [rad/s]  요 각속도 명령, 반시계 (왼쪽으로 돎) + / yaw-rate command, CCW (turning left) +
%   v_full [m/s]    throttle 400 count 일 때 궤도 속도 (0.20) / track speed at 400 counts of throttle
%   w_full [rad/s]  steer 400 count 일 때 요 각속도 (1.37) / yaw rate at 400 counts of steer
%   db_v, db_w [count]  ESC 데드밴드 역보상 크기 (47, 20) / ESC dead-band pre-compensation
% 출력 / Output
%   motor_pwm [2x1, count]  [왼쪽; 오른쪽] 서보 펄스 폭 [us] 와 같은 수, 1500 = 정지, 1100-1900
%                           [left; right] servo pulse width in microseconds, 1500 = stop, 1100-1900
%                           -> /motor_pwm (geometry_msgs/Point x, y) -> Arduino Mega -> C620 ESC
% 원리 / Principle
%   1) 실기에서는 PID 출력 (-0.5 ~ 0.5, 단위 없음) 이 V, W 로 들어간다. 1 판에는 내부 PID 가 없으므로
%      속도 명령을 같은 범위로 정규화: V = 0.5 v_cmd / v_full
%      The real model feeds PID outputs (-0.5 to 0.5, unitless) as V, W. v1 has no inner PID, so the
%      speed commands are normalised to the same range: V = 0.5 v_cmd / v_full
%   2) throttle = db tanh(V/0.02) + (400 - db) V/0.5 : 0 근처에서 db 만큼 뛰어 ESC 데드존을 건너뛴다
%      throttle jumps by db near zero to step over the ESC dead zone, then rises linearly to 400
%   3) left = throttle - steer, right = throttle + steer (steer > 0 이면 오른쪽이 빨라 왼쪽으로 돈다)
%      (steer > 0: the right track is faster, so the robot turns left)
%   4) 오른쪽 모터는 거울 대칭으로 달려 있어 부호를 뒤집는다 / the right motor is mirrored, so its sign is inverted
V = max(-0.5, min(0.5, 0.5 * v_cmd / v_full));
W = max(-0.5, min(0.5, 0.5 * w_cmd / w_full));
NEUTRAL = 1500;  MAX_OFFSET = 400;  V_EPS = 0.02;  W_EPS = 0.10;
db_v_c = max(0, min(MAX_OFFSET, db_v));
db_w_c = max(0, min(MAX_OFFSET, db_w));
throttle = db_v_c * tanh(V / V_EPS) + (MAX_OFFSET - db_v_c) * (V / 0.5);
steer    = db_w_c * tanh(W / W_EPS) + (MAX_OFFSET - db_w_c) * (W / 0.5);
left_raw  = throttle - steer;
right_raw = throttle + steer;
right_inv = -right_raw;                         % 우측 모터 물리적 반전 / right motor physically inverted
motor_pwm = [max(1100, min(1900, NEUTRAL + left_raw));
             max(1100, min(1900, NEUTRAL + right_inv))];

== matlab function XY_2_pen_ros2/PenCtrl/PenComp ==
  data: lineAB input; s_cmd output; mode input; pose input; pen_d input; stage_c input; pen_on output; sigma output
function [s_cmd, pen_on, sigma] = PenComp(lineAB, mode, pose, pen_d, stage_c)
% PenComp : 펜 기구학 보상. 펜이 직선 위에 오도록 스테이지 위치 명령을 계산한다
% PenComp : pen kinematic compensation. Computes the stage position command that puts the pen on the line
% 입력 / Inputs
%   lineAB  [4x1, m]   [A; B] 펜이 그릴 직선, 벽면 좌표 (x 오른쪽, y 위) / pen line in wall coordinates (x right, y up)
%   mode    [-]        미션 모드. 3 (직선 추종) 일 때만 보상 / mission mode; compensates only in mode 3
%   pose    [3x1: m, m, rad]  측정 태그 자세 [x; y; psi] (Nav) / measured tag pose
%   pen_d   [2x1, m]   태그 -> 펜 레버암, 바디 좌표 [x_B; y_B], 스테이지 중앙일 때 (= d)
%                      tag-to-pen lever arm in body axes, with the stage centred (= d)
%   stage_c [mm]       스테이지 중앙 (50.8, 두 축 같음) / stage centre (50.8 on both axes)
% 출력 / Outputs
%   s_cmd  [2x1, mm]   스테이지 목표 [X; Y] (X = x_B 전진 축, Y = y_B 왼쪽 축), 0-101.6
%                      stage target [X; Y] (X along x_B forward, Y along y_B left) -> /stage/target_pos
%   pen_on [0/1]       1 = 펜 다운 (펜 목표가 A 와 B 사이) / 1 = pen down (pen target between A and B)
%   sigma  [m]         직선 위 진행 거리 (A 에서 0, B 에서 L) / distance travelled along the line
% 원리 / Principle
%   펜 = 태그 + R(psi) (pen_d + (s - s_c)/1000) 을 s 에 대해 푼다. /1000 은 mm -> m.
%   Solve  pen = tag + R(psi) (pen_d + (s - s_c)/1000)  for s.  The 1000 converts m to mm.
%   p_des : 스테이지 중앙일 때 펜 위치 c0 를 직선에 내린 수선의 발
%           foot of the perpendicular from c0 (pen with the stage centred) to the line
%   진행 방향은 로봇이 맡고, 스테이지는 직선과의 어긋남(횡오차 + heading 오차)만 지운다
%   The robot provides the motion along the line; the stage removes only the offset from the line.
A = lineAB(1:2);  B = lineAB(3:4);
L = norm(B - A);  u = (B - A) / max(L, 1e-9);
pT = pose(1:2);
R  = [cos(pose(3)) -sin(pose(3)); sin(pose(3)) cos(pose(3))];
pc = pT + R * pen_d;                 % 스테이지 중앙일 때 펜 위치 / pen position with the stage centred
sigma = dot(u, pc - A);              % 직선 위 진행 거리 / distance along the line
pen_on = 0;
s_cmd = [stage_c; stage_c];
if round(mode) == 3
    % 직선 구간에 들어서면 펜을 내리기 전부터 스테이지를 미리 보낸다 (시작 과도 제거)
    % p_des 는 직선 위 수선의 발 (A, B 로 자르지 않는다): 진행 방향은 로봇이 맡고
    % 스테이지는 직선에서 벗어난 만큼만 지운다. A 로 자르면 펜이 A 앞에 있을 때
    % 남은 진행 거리(line_pre = 60 mm)까지 스테이지가 메우려 해서 행정 끝에 닿는다
%   On entering the line segment the stage is sent ahead even before pen down (removes the start transient).
%   p_des is the foot of the perpendicular on the line (not clipped to A, B): the robot provides the motion
%   along the line and the stage removes only the offset. Clipping to A would make the stage try to cover
%   the remaining run-in (line_pre = 60 mm) while the pen is before A, hitting the end of travel
    p_des = A + sigma * u;
    e_b = R' * (p_des - pT) - pen_d;   % 바디 좌표 펜 이동량 [m] / pen displacement in body frame [m]
    s_cmd = stage_c + 1000 * e_b;
    pen_on = double(sigma >= 0 && sigma <= L);
end

== matlab function XY_2_pen_ros2/Mission/Guards ==
  data: pose input; dist_start output; pen_A input; pen_B input; pen_d input; line_pre input; line_post input; r_tag input; th_err output; along_rem output
function [dist_start, th_err, along_rem] = Guards(pose, pen_A, pen_B, pen_d, line_pre, line_post, r_tag)
% Guards : Stateflow 전이 조건에 쓸 거리·각 (실기 Chart 의 dist, th_err, dist_to_WP2 와 같은 뜻)
% Guards : distances and angle used by the Stateflow transitions (dist, th_err, dist_to_WP2 of the real Chart)
% 입력 / Inputs
%   pose         [3x1: m, m, rad] 측정 태그 자세 [x; y; psi] / measured tag pose
%   pen_A, pen_B [2x1, m]   펜이 그릴 직선의 시작·끝 (벽면) / start and end of the pen line (wall)
%   pen_d        [2x1, m]   태그 -> 펜 레버암, 바디 좌표, 스테이지 중앙일 때 / tag-to-pen lever arm, body frame, stage centred
%   line_pre, line_post [m] 직선 앞뒤로 로봇이 더 가는 거리 / run-in and run-out lengths of the robot segment
%   r_tag        [2x1, m]   로봇 중심 -> 태그, 바디 좌표 / robot centre to tag, body frame
% 출력 / Outputs
%   dist_start [m]   추정 중심과 출발 중심 cA 의 거리 (모드 1 -> 2) / estimated centre to start centre cA (mode 1 -> 2)
%   th_err     [rad] 직선 방향 - heading, [-pi, pi] (모드 2 -> 3) / line direction minus heading (mode 2 -> 3)
%   along_rem  [m]   태그에서 로봇 끝점 rB 까지 남은 진행 거리 (모드 3 -> 4) / distance left to rB along the line (mode 3 -> 4)
th = atan2(pen_B(2) - pen_A(2), pen_B(1) - pen_A(1));   % 펜 직선 방향 / pen line direction
u  = [cos(th); sin(th)];
R  = [cos(th) -sin(th); sin(th) cos(th)];
% 로봇(태그)이 따라갈 선 = 펜 직선을 R*pen_d 만큼 옮긴 것 (스테이지 중앙일 때 펜이 직선 위)
% Line the robot (tag) follows = pen line shifted by R*pen_d (pen on the line when the stage is centred)
rA = pen_A - R*pen_d - u*line_pre;    % 로봇 출발점 (펜이 A 에 닿기 line_pre 전) / robot start (line_pre before the pen reaches A)
rB = pen_B - R*pen_d + u*line_post;   % 로봇 끝점 / robot end point
% 제자리 회전은 중심 둘레로 돈다: 회전 뒤 태그가 rA 에 오려면 중심이 cA 에 있어야 한다
% In-place turns pivot about the centre: for the tag to end at rA the centre must be at cA
cA = rA - R*r_tag;
p = pose(1:2);
Rp = [cos(pose(3)) -sin(pose(3)); sin(pose(3)) cos(pose(3))];
dist_start = norm(cA - (p - Rp*r_tag));                        % 중심과 출발 중심 cA 의 거리 / centre to start centre cA
th_err     = atan2(sin(th - pose(3)), cos(th - pose(3)));      % 직선 방향 오차 / line direction error
along_rem  = dot(rB - p, u);                                   % 끝점까지 남은 진행 거리 / distance left to the end point

== matlab function XY_2_pen_ros2/Nav/NavFcn ==
  settings: updateMethod=DISCRETE  sampleTime=Ts_ctrl
  data: zerokey_position input; pose output; zerokey_vel input; imu_quat input; psi0 input; tau_pred input; zk_xsign input
function pose = NavFcn(zerokey_position, zerokey_vel, imu_quat, psi0, tau_pred, zk_xsign)
% NavFcn : 센서 토픽 -> 측정 자세 (항법)
% NavFcn : sensor topics -> measured pose (navigation)
% 입력 / Inputs
%   zerokey_position [3x1, m]   /zerokey/position point.(x,y,z). 태그 월드 좌표: x 벽 수평, y 벽 법선, z 높이
%                               tag world position: x horizontal, y wall normal, z height
%   zerokey_vel      [3x1, m/s] /zerokey/vel twist.linear.(x,y,z). 태그 월드 속도 / tag world velocity
%   imu_quat         [4x1, -]   /imu/data orientation (w,x,y,z). Xsens 자세 쿼터니언 / Xsens attitude quaternion
%   psi0             [1, rad]   출발 heading (오른쪽 0, 천장 pi/2) / initial heading (0 = right, pi/2 = up)
%   tau_pred         [1, s]     ZeroKey 지연 보상 시간 (0 = 끔) / ZeroKey latency compensation (0 = off)
%   zk_xsign         [-1 / +1]  ZeroKey x 방향: -1 = 벽 정면에서 왼쪽 +, +1 = 오른쪽 + / ZeroKey x: -1 left +, +1 right +
% 출력 / Output
%   pose [3x1: m, m, rad]  [x; y; psi] = 태그 벽면 위치 (x 오른쪽 +, y 위 +) + heading (x 축에서 반시계)
%                          [x; y; psi] = tag position on the wall (x right, y up) + heading (CCW from x)
% 원리 / Principle
%   벽면 x = zk_xsign * ZeroKey x, 벽면 y = ZeroKey z (REP-103 형: z 가 벽 바깥인 오른손 좌표계).
%   철판 벽에서는 자력계를 못 쓰므로 heading 은 첫 유효 샘플의 요각을 0 으로 잡은 상대 요각에 psi0 를 더한 값이다.
%   Wall x = zk_xsign * ZeroKey x, wall y = ZeroKey z (REP-103 style, right-handed with z out of the wall).
%   The steel wall disturbs the magnetometer, so heading is the yaw relative to the first valid sample, plus psi0.
persistent yaw0 ok
if isempty(ok), ok = false; yaw0 = 0; end
qw = imu_quat(1); qx = imu_quat(2); qy = imu_quat(3); qz = imu_quat(4);
yaw = atan2(2*(qw*qz + qx*qy), 1 - 2*(qy*qy + qz*qz));
if ~ok && (abs(qw) + abs(qx) + abs(qy) + abs(qz)) > 0.5
    yaw0 = yaw;  ok = true;
end
a = yaw - yaw0 + psi0;
pose = [zk_xsign * zerokey_position(1); zerokey_position(3); atan2(sin(a), cos(a))];
% ZeroKey 지연 보상 (tau_pred = 0 이면 끔): 측정 속도로 tau_pred 만큼 앞으로 내다본다
% ZeroKey latency compensation (off when tau_pred = 0): predicts ahead by tau_pred with the measured velocity
pose(1:2) = pose(1:2) + tau_pred * [zk_xsign * zerokey_vel(1); zerokey_vel(3)];

== stateflow chart XY_2_pen_ros2/Mission/ModeChart ==
  settings: updateMethod=DISCRETE  sampleTime=Ts_ctrl
  state Goto_Start
    entry:
    mode = 1;
  state Turning
    entry:
    mode = 2;
  state Line_Tracking
    entry:
    mode = 3;
    t_line = t;
  state Stop_Destination
    entry:
    mode = 4;
  state Done
    entry:
    done = 1;
  (default) -> Goto_Start
  Goto_Start -> Turning : [dist_start < d_reach]
  Turning -> Line_Tracking : after(1.0,sec)[abs(th_err) < th_tol]
  Line_Tracking -> Stop_Destination : [along_rem < d_reach]
  Stop_Destination -> Done : after(2.0,sec)
  data: dist_start input; th_err input; along_rem input; t input; mode output double =1; t_line output double =0; done output double =0; d_reach parameter; th_tol parameter

== matlab function XY_2_pen_ros2/Mission/Waypoints ==
  data: mode input; WP_prev output; pen_A input; pen_B input; pen_d input; line_pre input; line_post input; r_tag input; WP_target output; lineAB output
function [WP_prev, WP_target, lineAB] = Waypoints(mode, pen_A, pen_B, pen_d, line_pre, line_post, r_tag)
% Waypoints : 모드에 따라 로봇이 따라갈 선분을 낸다 (6WP waypoint_manager 역할)
% Waypoints : gives the segment the robot follows in each mode (role of the 6WP waypoint_manager)
% 입력 / Inputs
%   mode [-]  1 출발점 이동, 2 회전, 3 직선 추종, 4 정지, 5 종료 / 1 go to start, 2 turn, 3 line, 4 stop, 5 done
%   pen_A, pen_B, pen_d, line_pre, line_post, r_tag : Guards 와 같음 / same as Guards
% 출력 / Outputs
%   WP_prev   [2x1, m] 태그 선분 시작 rA (펜이 A 에 닿기 line_pre 전) / tag segment start rA
%   WP_target [2x1, m] 모드 1: 출발 중심 cA (중심 기준), 그 뒤: 태그 선분 끝 rB
%                      mode 1: start centre cA (centre-referenced); afterwards: tag segment end rB
%   lineAB    [4x1, m] [A; B] 펜 직선 (PenComp 로 간다) / pen line, sent to PenComp
% 원리 / Principle
%   스테이지가 중앙일 때 펜이 직선 위에 오도록, 태그가 갈 선분은 펜 직선을 R(theta_l) pen_d 만큼 옮긴 것이다.
%   The tag segment is the pen line shifted by -R(theta_l) pen_d, so that the pen is on the line when the stage is centred.
th = atan2(pen_B(2) - pen_A(2), pen_B(1) - pen_A(1));   % 펜 직선 방향 / pen line direction
u  = [cos(th); sin(th)];
R  = [cos(th) -sin(th); sin(th) cos(th)];
% 로봇(태그)이 따라갈 선 = 펜 직선을 R*pen_d 만큼 옮긴 것 (스테이지 중앙일 때 펜이 직선 위)
% Line the robot (tag) follows = pen line shifted by R*pen_d (pen on the line when the stage is centred)
rA = pen_A - R*pen_d - u*line_pre;    % 로봇 출발점 (펜이 A 에 닿기 line_pre 전) / robot start (line_pre before the pen reaches A)
rB = pen_B - R*pen_d + u*line_post;   % 로봇 끝점 / robot end point
% 제자리 회전은 중심 둘레로 돈다: 회전 뒤 태그가 rA 에 오려면 중심이 cA 에 있어야 한다
% In-place turns pivot about the centre: for the tag to end at rA the centre must be at cA
cA = rA - R*r_tag;
WP_prev = rA;
if round(mode) <= 1
    WP_target = cA;
else
    WP_target = rB;
end
lineAB = [pen_A; pen_B];

== matlab function XY_2_pen_ros2/RobotCtrl/M1_GotoStart/Fcn1_GotoStart ==
  data: WP_target input; v output; pose input; K_dist input; K_yaw input; r_tag input; w output
function [v, w] = Goto_Start_Position(WP_target, pose, K_dist, K_yaw, r_tag)
% 모드 1 : 6WP_sim Goto_Start_Position, Method 2 (리아프노프형). 6WP 와 같이 로봇 중심을 목표로 보낸다
% Mode 1 : 6WP_sim Goto_Start_Position, Method 2. Drives the robot centre (as in 6WP_sim) to the target
% 입력 / Inputs
%   WP_target [2x1, m]   출발 중심 cA (벽면) / start centre cA (wall)
%   pose      [3x1: m, m, rad] 측정 태그 자세 / measured tag pose
%   K_dist    [1/s]  거리 게인 / distance gain;   K_yaw [1/s]  방향 게인 / bearing gain
%   r_tag     [2x1, m]  중심 -> 태그 (바디) / centre to tag (body)
% 출력 / Outputs
%   v [m/s]   전진 속도 명령 / forward speed command;   w [rad/s] 요 각속도 명령 (반시계 +) / yaw-rate command (CCW +)
% 원리 / Principle
%   v = K_dist rho max(0, cos a), w = K_yaw a + 0.5 sin a cos a. a = 목표 방위 - heading.
%   방향이 90 도 넘게 틀리면 서서 돌기만 한다 / turns on the spot while the bearing error exceeds 90 deg
c = pose(1:2) - [cos(pose(3)) -sin(pose(3)); sin(pose(3)) cos(pose(3))] * r_tag;   % 중심 추정 / centre estimate
err_x = WP_target(1) - c(1);  err_y = WP_target(2) - c(2);
dist = hypot(err_x, err_y);
target_th = atan2(err_y, err_x);
a = atan2(sin(target_th - pose(3)), cos(target_th - pose(3)));
v = K_dist * dist * max(0, cos(a));            % 방향이 맞을 때만 전진 / forward only when roughly aligned
w = K_yaw * a + 0.5 * sin(a) * cos(a);         % 비선형 감쇠항 / nonlinear damping term

== matlab function XY_2_pen_ros2/RobotCtrl/M2_Turn/Fcn2_Turn ==
  data: WP_prev input; v output; WP_target input; pose input; K_yaw input; w output
function [v, w] = Turning_Straight_Mode(WP_prev, WP_target, pose, K_yaw)
% 모드 2 : 6WP_sim Turning_Straight_Mode — 제자리 회전으로 heading 을 직선 방향에 맞춘다
% Mode 2 : 6WP_sim Turning_Straight_Mode — turns on the spot until the heading matches the line
% 입력 / Inputs
%   WP_prev, WP_target [2x1, m] 태그 선분 rA, rB / tag segment;  pose [m, m, rad];  K_yaw [1/s]
% 출력 / Outputs
%   v = 0 [m/s],  w = K_yaw wrap(theta_l - psi) [rad/s]
th_final = atan2(WP_target(2) - WP_prev(2), WP_target(1) - WP_prev(1));
th_err = atan2(sin(th_final - pose(3)), cos(th_final - pose(3)));
v = 0;
w = K_yaw * th_err;
